simulink model "ASM_Traffic_A11"  (R2026a)
settings: Solver=ode1  StartTime=SIM.tstart.v  StopTime=SIM.tend.v  FixedStep=SIM.StepSize.v
PostLoadFcn:
  | if any(exist('dsrtsu_mdlpostloadfcn', 'file') ~= 0), dsrtsu_mdlpostloadfcn('Execute', bdroot); end
  | try, asm_mdl_postloadfcn(bdroot, 'UpdateModel', 3600); catch, disp(lasterr); end,
InitFcn:
  | , if any(exist('rtifpga_mdlclblib', 'file') ~= 0), rtifpga_mdlclblib('Init', bdroot); end,
  | , if any(exist('dsmpb_private', 'file') ~= 0), dsmpb_private('dsmpb_mdlclblib', 'Init', bdroot); end,
undefined symbols (not defined in the file): _to_, a0b2, ASM_BrakeHydraulics_DemoSystems, ASM_VehicleDynamics_DemoSystems, b98103fe8ad365046cd0, BrakeCircuit, controllerConfig, CPT, Crankshaft, DiscIntNeverNeededParam, dsmsi, FinalDriveAssembly, instance, MDL, ModeSignals, mu, Pos_BrakePedal_Maneuver, rad, RefSignals, s_to_rpm, SIM, SoftECU, Suspension, Tire, Transmission
libraries: ASM_Traffic_lib x135, simulink x98, ASM_Utils_lib x77, ASM_VehicleDynamics_lib x70, ASM_Environment_lib x22, dsmpblib x20, dsmsilib x15, MDLD_Utils_lib x10, ASM_BrakeHydraulics_lib x3, sl_discontinuities x2
(part 11 of 63)

== system ASM_Traffic_A11/Drivetrain/Control/SoftECU_Drivetrain ==
  note: -------------
  note: Plant
  note: -------------
  note: User Interface
  note: Control
  note: -------------
  note: Inport colors:
  note: External Signals
  note: -------------
  UserInterface : Inport
  Interface_In : Inport  Port=2
  Plant : Inport  Port=3
  Bus Creator : BusCreator  Inputs=8
  Bus Selector1 : BusSelector  OutputSignals=ExternalModel.Pos_AccPedal[%],ExternalModel.SelectorLever[-3T|-2P|-1R|0N|1D],ExternalModel.Sw_TipShift[-1Down|0Off|1Up],ExternalModel.Gear_Max[0Off|1_n],ExternalModel.Reset_States[0|1],ExternalModel.Gear_Maneuver[],ExternalModel.Mode_GearClutch[1Stim|2Driver|3OpenClutch|4RefGear],ExternalModel.State_Engine[0|1|2|3|4],ExternalModel.State_StartStop[1Off|2NotReady|3Ready|4EngStopped],ExternalModel.Enable_v_Init[0|1]
  Bus Selector7 : BusSelector  OutputSignals=Drivetrain.Crankshaft.n_Engine[rad|s],Drivetrain.Transmission.OutputSignals.omega_In_Trm[rad|s],Drivetrain.Transmission.OutputSignals.omega_Out_Trm[rad|s],Drivetrain.Transmission.OutputSignals.Gear[]
  Constant{,1..3} (4 alike) : Constant  Value=0
  ModelDesk_MC_ID_SoftECU : ASM_Utils_lib/ModelDeskInterface/ModelDesk_MC  Tag=ASM_MAINCOMPONENT  Editable=off  MainComponent=SoftECU
  SoftECU_Transmission : Subsystem
  Terminator_1 : Terminator
  ASMSignalBus : Outport  VectorParamsAs1DForOutWhenUnconnected=off
  Out : Outport  Port=2  VectorParamsAs1DForOutWhenUnconnected=off
  wires:
  Bus Selector1/9 -> SoftECU_Transmission/13(State_StartStop[1Off|2NotReady|3Ready|4EngStopped])  "<State_StartStop[1Off|2NotReady|3Ready|4EngStopped]>"
  Bus Selector1/7 -> SoftECU_Transmission/11(GearClutch_Mode[1Stim|2SoftECU|3OpenClutch|4RefGear])  "<Mode_GearClutch[1Stim|2Driver|3OpenClutch|4RefGear]>"
  Bus Selector1/6 -> SoftECU_Transmission/10(Gear_Maneuver[])  "<Gear_Maneuver[]>"
  Bus Selector1/5 -> SoftECU_Transmission/9(Reset[0|1])  "<Reset_States[0|1]>"
  Bus Selector1/4 -> SoftECU_Transmission/8(Gear_Max_Maneuver[0Off|1_n])  "<Gear_Max[0Off|1_n]>"
  Bus Selector1/3 -> SoftECU_Transmission/7(TipShift[-1Down|0Off|1Up])  "<Sw_TipShift[-1Down|0Off|1Up]>"
  Bus Selector1/2 -> SoftECU_Transmission/6(SelectorLever[-3T|-2P|-1R|0N|1D])  "<SelectorLever[-3T|-2P|-1R|0N|1D]>"
  Bus Selector1/1 -> SoftECU_Transmission/5(Pos_AccPedal_Driver[%])  "<Pos_AccPedal[%]>"
  Bus Selector1/8 -> SoftECU_Transmission/12(State_Engine[0|1|2|3|4])  "<State_Engine[0|1|2|3|4]>"
  Interface_In/1 -> Bus Selector1/1
  Constant3/1 -> Bus Creator/8  "Ctrl_Clutch_4WD[0_1]"
  Constant2/1 -> Bus Creator/7  "Ctrl_RearDiff[0_1]"
  Constant1/1 -> Bus Creator/6  "Ctrl_FrontDiff[0_1]"
  Constant/1 -> Bus Creator/5  "Ctrl_CentralDiff[0_1]"
  UserInterface/1 -> Terminator_1/1
  Bus Creator/1 -> Out/1  "Drivetrain"
  SoftECU_Transmission/5(Gear[]) -> Bus Creator/4  "Gear[]"
  SoftECU_Transmission/4(Ctrl_Lockup_Clutch[0_1]) -> Bus Creator/3  "Ctrl_Lockup_Clutch[0_1]"
  SoftECU_Transmission/3(Ctrl_Parking_Pawl[0|1]) -> Bus Creator/2  "Ctrl_Parking_Pawl[0|1]"
  SoftECU_Transmission/2(Factor_Trq_Engine_Red[%]) -> Bus Creator/1  "Factor_Trq_Engine_Red[%]"
  Bus Selector7/4 -> SoftECU_Transmission/4(Gear_Current[])  "<Gear[]>"
  Bus Selector7/3 -> SoftECU_Transmission/3(omega_Out_Trm[rad|s])  "<omega_Out_Trm[rad|s]>"
  Bus Selector7/2 -> SoftECU_Transmission/2(omega_In_Trm[rad|s])  "<omega_In_Trm[rad|s]>"
  Bus Selector7/1 -> SoftECU_Transmission/1(n_Engine[rad|s])  "<n_Engine[rad|s]>"
  Plant/1 -> Bus Selector7/1
  SoftECU_Transmission/1(ASMSignalBus) -> ASMSignalBus/1
  Bus Selector1/10 -> SoftECU_Transmission/14(Enable_v_Init[0|1])  "<Enable_v_Init[0|1]>"

== system ASM_Traffic_A11/Drivetrain/Control/Sw_ECU_Signals ==
  SoftECU : Inport
  ExternalECU : Inport  Port=2
  Bus Creator4 : BusCreator  Inputs=8
  Bus Selector1 : BusSelector  OutputSignals=ExternalECU.Factor_Trq_Engine_Red[%],ExternalECU.Ctrl_Parking_Pawl[0|1],ExternalECU.Ctrl_Lockup_Clutch[0_1],ExternalECU.Gear[],ExternalECU.Ctrl_CentralDiff[0_1],ExternalECU.Ctrl_FrontDiff[0_1],ExternalECU.Ctrl_RearDiff[0_1],ExternalECU.Ctrl_Clutch_4WD[0_1]
  Bus Selector2 : BusSelector  OutputSignals=Factor_Trq_Engine_Red[%],Ctrl_Parking_Pawl[0|1],Ctrl_Lockup_Clutch[0_1],Gear[],Ctrl_CentralDiff[0_1],Ctrl_FrontDiff[0_1],Ctrl_RearDiff[0_1],Ctrl_Clutch_4WD[0_1]
  Ctrl_CentralDiff[0_1] : Subsystem
  Ctrl_Clutch_4WD[0_1] : Subsystem
  Ctrl_FrontDiff[0_1] : Subsystem
  Ctrl_Lockup_Clutch[0_1] : Subsystem
  Ctrl_Parking_Pawl[0|1] : Subsystem
  Ctrl_RearDiff[0_1] : Subsystem
  Factor_Trq_Engine_Red[%] : Subsystem
  Gear[] : Subsystem
  ECU_Signals : Outport  VectorParamsAs1DForOutWhenUnconnected=off
  wires:
  Ctrl_Clutch_4WD[0_1]/1(Ctrl_Clutch_4WD[0_1]) -> Bus Creator4/8  "Ctrl_Clutch_4WD[0_1]"
  Ctrl_RearDiff[0_1]/1(Ctrl_RearDiff[0_1]) -> Bus Creator4/7  "Ctrl_RearDiff[0_1]"
  Ctrl_FrontDiff[0_1]/1(Ctrl_FrontDiff[0_1]) -> Bus Creator4/6  "Ctrl_FrontDiff[0_1]"
  Ctrl_CentralDiff[0_1]/1(Ctrl_CentralDiff[0_1]) -> Bus Creator4/5  "Ctrl_CentralDiff[0_1]"
  Gear[]/1(Gear[]) -> Bus Creator4/4  "Gear[]"
  Ctrl_Lockup_Clutch[0_1]/1(Ctrl_Lockup_Clutch[0_1]) -> Bus Creator4/3  "Ctrl_Lockup_Clutch[0_1]"
  Ctrl_Parking_Pawl[0|1]/1(Ctrl_Parking_Pawl[0|1]) -> Bus Creator4/2  "Ctrl_Parking_Pawl[0|1]"
  Factor_Trq_Engine_Red[%]/1(Factor_Trq_Engine_Red[%]) -> Bus Creator4/1  "Factor_Trq_Engine_Red[%]"
  Bus Selector1/4 -> Gear[]/2(RealECU)  "<Gear[]>"
  Bus Selector1/5 -> Ctrl_CentralDiff[0_1]/2(RealECU)  "<Ctrl_CentralDiff[0_1]>"
  Bus Selector1/6 -> Ctrl_FrontDiff[0_1]/2(RealECU)  "<Ctrl_FrontDiff[0_1]>"
  Bus Selector1/7 -> Ctrl_RearDiff[0_1]/2(RealECU)  "<Ctrl_RearDiff[0_1]>"
  Bus Selector1/8 -> Ctrl_Clutch_4WD[0_1]/2(RealECU)  "<Ctrl_Clutch_4WD[0_1]>"
  Bus Selector1/3 -> Ctrl_Lockup_Clutch[0_1]/2(RealECU)  "<Ctrl_Lockup_Clutch[0_1]>"
  Bus Selector1/2 -> Ctrl_Parking_Pawl[0|1]/2(RealECU)  "<Ctrl_Parking_Pawl[0|1]>"
  Bus Selector1/1 -> Factor_Trq_Engine_Red[%]/2(RealECU)  "<Factor_Trq_Engine_Red[%]>"
  Bus Selector2/8 -> Ctrl_Clutch_4WD[0_1]/1(SoftECU)  "<Ctrl_Clutch_4WD[0_1]>"
  Bus Selector2/7 -> Ctrl_RearDiff[0_1]/1(SoftECU)  "<Ctrl_RearDiff[0_1]>"
  Bus Selector2/6 -> Ctrl_FrontDiff[0_1]/1(SoftECU)  "<Ctrl_FrontDiff[0_1]>"
  Bus Selector2/5 -> Ctrl_CentralDiff[0_1]/1(SoftECU)  "<Ctrl_CentralDiff[0_1]>"
  Bus Selector2/4 -> Gear[]/1(SoftECU)  "<Gear[]>"
  Bus Selector2/3 -> Ctrl_Lockup_Clutch[0_1]/1(SoftECU)  "<Ctrl_Lockup_Clutch[0_1]>"
  Bus Selector2/2 -> Ctrl_Parking_Pawl[0|1]/1(SoftECU)  "<Ctrl_Parking_Pawl[0|1]>"
  Bus Selector2/1 -> Factor_Trq_Engine_Red[%]/1(SoftECU)  "<Factor_Trq_Engine_Red[%]>"
  Bus Creator4/1 -> ECU_Signals/1  "Control"
  SoftECU/1 -> Bus Selector2/1
  ExternalECU/1 -> Bus Selector1/1

== system ASM_Traffic_A11/Drivetrain/Control/UserInterface ==
  note: Drivetrain Control
  In : Inport
  ASMSignalBus_Control : Subsystem
  DISP_Control : Subsystem
  PAR_Control : Subsystem
  Out : Outport  VectorParamsAs1DForOutWhenUnconnected=off
  wires:
  PAR_Control/1(Out) -> Out/1
  In/1 -> DISP_Control/1(In), ASMSignalBus_Control/1(In)

== system ASM_Traffic_A11/Drivetrain/Interface_In/ExternalSignals ==
  Enable : EnablePort
  ExternalECU_Transmission : Subsystem
  ExternalECU_Transmission_In : dsmpblib/Data Inport  Tag=ASM_MPB  Priority=10000
      settings: SourceProductName=dSPACE Model Interface Package for Simulink (MIPS)
  ExternalECU_Transmission_Out : Outport
  wires:
  ExternalECU_Transmission/1(Out) -> ExternalECU_Transmission_Out/1
  ExternalECU_Transmission_In/8 -> ExternalECU_Transmission/8(Ctrl_Clutch_4WD[0_1])
  ExternalECU_Transmission_In/7 -> ExternalECU_Transmission/7(Ctrl_RearDiff[0_1])
  ExternalECU_Transmission_In/6 -> ExternalECU_Transmission/6(Ctrl_FrontDiff[0_1])
  ExternalECU_Transmission_In/5 -> ExternalECU_Transmission/5(Ctrl_CentralDiff[0_1])
  ExternalECU_Transmission_In/4 -> ExternalECU_Transmission/4(Gear[])
  ExternalECU_Transmission_In/3 -> ExternalECU_Transmission/3(Ctrl_Lockup_Clutch[0_1])
  ExternalECU_Transmission_In/2 -> ExternalECU_Transmission/2(Ctrl_Parking_Pawl[0|1])
  ExternalECU_Transmission_In/1 -> ExternalECU_Transmission/1(Factor_Trq_Engine_Red[%])

== system ASM_Traffic_A11/Drivetrain/Interface_In/ModelSignals ==
  Sw_ModelPortBlocks[0Disabled|1Enabled] : Inport
  Sw_ModelDeskPlottingInterface[0Disabled|1Enabled] : Inport  Port=2
  n_Engine_Set[rpm] : Inport  Port=3
  Sw_Testbench[0Off|1On] : Inport  Port=4
  Pos_ClutchPedal[%] : Inport  Port=5
  Gear[] : Inport  Port=6
  Reset_States[0|1] : Inport  Port=7
  Trq_MeanEff_Engine[Nm] : Inport  Port=8
  omega_Wheel[FL;FR;RL;RR][rad|s] : Inport  Port=9
  Enable_v_Init[0|1] : Inport  Port=10
  Pos_AccPedal[%] : Inport  Port=11
  SelectorLever[-3T|-2P|-1R|0N|1D] : Inport  Port=12  PortDimensions=1
  Sw_TipShift[-1Down|0Off|1Up] : Inport  Port=13
  Gear_Maneuver[] : Inport  Port=14
  Mode_GearClutch[1Stim|2Driver|3OpenClutch|4RefGear] : Inport  Port=15
  Gear_Max[0Off|1_n] : Inport  Port=16
  State_Engine[0|1|2|3|4] : Inport  Port=17
  State_StartStop[1Off|2NotReady|3Ready|4EngStopped] : Inport  Port=18
  Sw_Starter[0|1] : Inport  Port=19
  CrankAngle_Cyl[aTDC] : Inport  Port=20
  Type_Engine_1[0Unkown|1Other|2Otto|3Diesel|4Electric] : Inport  Port=21
  Bus Creator : BusCreator  Inputs=21
  CrankAngle_Cyl[aTDC]_ : Subsystem
      mask Display: disp('')
  Enable_v_Init[0|1]_ : Subsystem
      mask Display: disp('')
  Gear[]_ : Subsystem
      mask Display: disp('')
  Gear_Maneuver[]_ : Subsystem
      mask Display: disp('')
  Gear_Max[0Off|1_n]_ : Subsystem
      mask Display: disp('')
  Mode_GearClutch[1Stim|2Driver|3OpenClutch|4RefGear]_ : Subsystem
      mask Display: disp('')
  Pos_AccPedal[%]_ : Subsystem
      mask Display: disp('')
  Pos_ClutchPedal[%]_ : Subsystem
      mask Display: disp('')
  Reset_States[0|1]_ : Subsystem
      mask Display: disp('')
  SelectorLever[-3T|-2P|-1R|0N|1D]_ : Subsystem
      mask Display: disp('')
  State_Engine[0|1|2|3|4]_ : Subsystem
      mask Display: disp('')
  State_StartStop[1Off|2NotReady|3Ready|4EngStopped]_ : Subsystem
      mask Display: disp('')
  Sw_ModelDeskPlottingInterface[0Disabled|1Enabled]_ : Subsystem
  Sw_ModelPortBlocks[0Disabled|1Enabled]_ : Subsystem
  Sw_Starter[0|1]_ : Subsystem
      mask Display: disp('')
  Sw_Testbench[0Off|1On]_ : Subsystem
      mask Display: disp('')
  Sw_TipShift[-1Down|0Off|1Up]_ : Subsystem
      mask Display: disp('')
  Trq_MeanEff_Engine[Nm]_ : Subsystem
      mask Display: disp('')
  Type_Engine_1[0Unkown|1Other|2Otto|3Diesel|4Electric]_ : Subsystem
      mask Display: disp('')
  n_Engine_Set[rpm]_ : Subsystem
      mask Display: disp('')
  omega_Wheel[FL;FR;RL;RR][rad|s]_ : Subsystem
      mask Display: disp('')
  Out : Outport  VectorParamsAs1DForOutWhenUnconnected=off
  wires:
  Sw_ModelDeskPlottingInterface[0Disabled|1Enabled]_/1(Out1) -> Bus Creator/2  "Sw_ModelDeskPlottingInterface[0Disabled|1Enabled]"
  Sw_ModelPortBlocks[0Disabled|1Enabled]_/1(Out1) -> Bus Creator/1  "Sw_ModelPortBlocks[0Disabled|1Enabled]"
  Sw_ModelDeskPlottingInterface[0Disabled|1Enabled]/1 -> Sw_ModelDeskPlottingInterface[0Disabled|1Enabled]_/1(In1)
  Sw_ModelPortBlocks[0Disabled|1Enabled]/1 -> Sw_ModelPortBlocks[0Disabled|1Enabled]_/1(In1)
  Bus Creator/1 -> Out/1  "ExternalModel"
  Pos_ClutchPedal[%]_/1(Out1) -> Bus Creator/5  "Pos_ClutchPedal[%]"
  Gear[]_/1(Out1) -> Bus Creator/6  "Gear[]"
  Gear[]/1 -> Gear[]_/1(In1)
  Pos_ClutchPedal[%]/1 -> Pos_ClutchPedal[%]_/1(In1)
  Sw_Testbench[0Off|1On]_/1(Out1) -> Bus Creator/4  "Sw_Testbench[0Off|1On]"
  Sw_Testbench[0Off|1On]/1 -> Sw_Testbench[0Off|1On]_/1(In1)
  n_Engine_Set[rpm]_/1(Out1) -> Bus Creator/3  "n_Engine_Set[rpm]"
  n_Engine_Set[rpm]/1 -> n_Engine_Set[rpm]_/1(In1)
  Reset_States[0|1]_/1(Out1) -> Bus Creator/7  "Reset_States[0|1]"
  Reset_States[0|1]/1 -> Reset_States[0|1]_/1(In1)
  Trq_MeanEff_Engine[Nm]_/1(Out1) -> Bus Creator/8  "Trq_MeanEff_Engine[Nm]"
  Trq_MeanEff_Engine[Nm]/1 -> Trq_MeanEff_Engine[Nm]_/1(In1)
  omega_Wheel[FL;FR;RL;RR][rad|s]_/1(Out1) -> Bus Creator/9  "omega_Wheel[FL;FR;RL;RR][rad|s]"
  omega_Wheel[FL;FR;RL;RR][rad|s]/1 -> omega_Wheel[FL;FR;RL;RR][rad|s]_/1(In1)
  Enable_v_Init[0|1]/1 -> Enable_v_Init[0|1]_/1(In1)
  Enable_v_Init[0|1]_/1(Out1) -> Bus Creator/10  "Enable_v_Init[0|1]"
  Sw_TipShift[-1Down|0Off|1Up]_/1(Out1) -> Bus Creator/13  "Sw_TipShift[-1Down|0Off|1Up]"
  Gear_Maneuver[]_/1(Out1) -> Bus Creator/14  "Gear_Maneuver[]"
  Pos_AccPedal[%]/1 -> Pos_AccPedal[%]_/1(In1)
  SelectorLever[-3T|-2P|-1R|0N|1D]/1 -> SelectorLever[-3T|-2P|-1R|0N|1D]_/1(In1)
  Mode_GearClutch[1Stim|2Driver|3OpenClutch|4RefGear]_/1(Out1) -> Bus Creator/15  "Mode_GearClutch[1Stim|2Driver|3OpenClutch|4RefGear]"
  Mode_GearClutch[1Stim|2Driver|3OpenClutch|4RefGear]/1 -> Mode_GearClutch[1Stim|2Driver|3OpenClutch|4RefGear]_/1(In1)
  Gear_Max[0Off|1_n]/1 -> Gear_Max[0Off|1_n]_/1(In1)
  Gear_Maneuver[]/1 -> Gear_Maneuver[]_/1(In1)
  Gear_Max[0Off|1_n]_/1(Out1) -> Bus Creator/16  "Gear_Max[0Off|1_n]"
  State_Engine[0|1|2|3|4]_/1(Out1) -> Bus Creator/17  "State_Engine[0|1|2|3|4]"
  Sw_TipShift[-1Down|0Off|1Up]/1 -> Sw_TipShift[-1Down|0Off|1Up]_/1(In1)
  State_StartStop[1Off|2NotReady|3Ready|4EngStopped]_/1(Out1) -> Bus Creator/18  "State_StartStop[1Off|2NotReady|3Ready|4EngStopped]"
  SelectorLever[-3T|-2P|-1R|0N|1D]_/1(Out1) -> Bus Creator/12  "SelectorLever[-3T|-2P|-1R|0N|1D]"
  Pos_AccPedal[%]_/1(Out1) -> Bus Creator/11  "Pos_AccPedal[%]"
  State_StartStop[1Off|2NotReady|3Ready|4EngStopped]/1 -> State_StartStop[1Off|2NotReady|3Ready|4EngStopped]_/1(In1)
  State_Engine[0|1|2|3|4]/1 -> State_Engine[0|1|2|3|4]_/1(In1)
  Sw_Starter[0|1]/1 -> Sw_Starter[0|1]_/1(In1)
  CrankAngle_Cyl[aTDC]/1 -> CrankAngle_Cyl[aTDC]_/1(In1)
  CrankAngle_Cyl[aTDC]_/1(Out1) -> Bus Creator/20  "CrankAngle_Cyl[aTDC]"
  Sw_Starter[0|1]_/1(Out1) -> Bus Creator/19  "Sw_Starter[0|1]"
  Type_Engine_1[0Unkown|1Other|2Otto|3Diesel|4Electric]_/1(Out1) -> Bus Creator/21  "Type_Engine_1[0Unkown|1Other|2Otto|3Diesel|4Electric]"
  Type_Engine_1[0Unkown|1Other|2Otto|3Diesel|4Electric]/1 -> Type_Engine_1[0Unkown|1Other|2Otto|3Diesel|4Electric]_/1(In1)

== system ASM_Traffic_A11/Drivetrain/Interface_Out/Animation ==
  n_Engine[rpm] : Inport
  Gear[] : Inport  Port=2
  BusCreator : BusCreator  Inputs=2
  Gear[]_ : Subsystem
      mask Display: disp('')
  n_Engine[rpm]_ : Subsystem
      mask Display: disp('')
  Out : Outport  VectorParamsAs1DForOutWhenUnconnected=off
  wires:
  BusCreator/1 -> Out/1  "Animation"
  n_Engine[rpm]_/1(Out1) -> BusCreator/1  "n_Engine[rpm]"
  Gear[]_/1(Out1) -> BusCreator/2  "Gear[]"
  n_Engine[rpm]/1 -> n_Engine[rpm]_/1(In1)
  Gear[]/1 -> Gear[]_/1(In1)

== system ASM_Traffic_A11/Drivetrain/Interface_Out/Control_ModelSignals ==
  Factor_Trq_Engine_Red[%] : Inport
  Ctrl_Parking_Pawl[0|1] : Inport  Port=2
  Bus Creator : BusCreator  Inputs=2
  Ctrl_Parking_Pawl[0|1]_ : Subsystem
      mask Display: disp('')
  Factor_Trq_Engine_Red[%]_ : Subsystem
      mask Display: disp('')
  Out : Outport  VectorParamsAs1DForOutWhenUnconnected=off
  wires:
  Factor_Trq_Engine_Red[%]/1 -> Factor_Trq_Engine_Red[%]_/1(In1)
  Bus Creator/1 -> Out/1  "Control"
  Factor_Trq_Engine_Red[%]_/1(Out1) -> Bus Creator/1  "Factor_Trq_Engine_Red[%]"
  Ctrl_Parking_Pawl[0|1]_/1(Out1) -> Bus Creator/2  "Ctrl_Parking_Pawl[0|1]"
  Ctrl_Parking_Pawl[0|1]/1 -> Ctrl_Parking_Pawl[0|1]_/1(In1)

== system ASM_Traffic_A11/Drivetrain/Interface_Out/Plant_ModelSignals ==
  n_Engine[rpm] : Inport
  omega_Out_Trm[rad|s] : Inport  Port=2
  Gear[] : Inport  Port=3
  i_FinalDrive[] : Inport  Port=4
  i_FrontDrive[] : Inport  Port=5
  i_RearDrive[] : Inport  Port=6
  TrqDistri_Front_Rear[0_1] : Inport  Port=7
  Trq_Out_Front_Diff[Nm] : Inport  Port=8
  Trq_Shaft[FL;FR;RL;RR][Nm] : Inport  Port=9
  i_unsync_Trm[] : Inport  Port=10
  Sw_CrankShaft_Reset[0Disabled|1Enabled] : Inport  Port=11
  Mode_Transmission[1Manual|2Automatic] : Inport  Port=12
  Mode_Drivetrain[1|2|3|4|5] : Inport  Port=13
  Type_Engine_1[0Unkown|1Other|2Otto|3Diesel|4Electric] : Inport  Port=14
  Trq_Engine_1[Nm] : Inport  Port=15
  n_Engine_1[rpm] : Inport  Port=16
  Type_Engine_2[0Unkown|1Other|2Otto|3Diesel|4Electric] : Inport  Port=17
  Trq_Engine_2[Nm] : Inport  Port=18
  n_Engine_2[rpm] : Inport  Port=19
  Trq_BSG[Nm] : Inport  Port=20
  Bus Creator : BusCreator  Inputs=20
  Gear[]_ : Subsystem
      mask Display: disp('')
  Mode_Drivetrain[1|2|3|4|5]_ : Subsystem
      mask Display: disp('')
  Mode_Transmission[1Manual|2Automatic]_ : Subsystem
      mask Display: disp('')
  Sw_CrankShaft_Reset[0Disabled|1Enabled]_ : Subsystem
      mask Display: disp('')
  TrqDistri_Front_Rear[0_1]_ : Subsystem
      mask Display: disp('')
  Trq_BSG[Nm]_ : Subsystem
      mask Display: disp('')
  Trq_Engine_1[Nm]_ : Subsystem
      mask Display: disp('')
  Trq_Engine_2[Nm]_ : Subsystem
      mask Display: disp('')
  Trq_Out_Front_Diff[Nm]_ : Subsystem
      mask Display: disp('')
  Trq_Shaft[FL;FR;RL;RR][Nm]_ : Subsystem
      mask Display: disp('')
  Type_Engine_1[0Unkown|1Other|2Otto|3Diesel|4Electric]_ : Subsystem
      mask Display: disp('')
  Type_Engine_2[0Unkown|1Other|2Otto|3Diesel|4Electric]_ : Subsystem
      mask Display: disp('')
  i_FinalDrive[]_ : Subsystem
      mask Display: disp('')
  i_FrontDrive[]_ : Subsystem
      mask Display: disp('')
  i_RearDrive[]_ : Subsystem
      mask Display: disp('')
  i_unsync_Trm[]_ : Subsystem
      mask Display: disp('')
  n_Engine[rpm]_ : Subsystem
      mask Display: disp('')
  n_Engine_1[rpm]_ : Subsystem
      mask Display: disp('')
  n_Engine_2[rpm]_ : Subsystem
      mask Display: disp('')
  omega_Out_Trm[rad|s]_ : Subsystem
      mask Display: disp('')
  Out : Outport  VectorParamsAs1DForOutWhenUnconnected=off
  wires:
  n_Engine_2[rpm]_/1(Out1) -> Bus Creator/19  "n_Engine_2[rpm]"
  n_Engine_2[rpm]/1 -> n_Engine_2[rpm]_/1(In1)
  n_Engine_1[rpm]_/1(Out1) -> Bus Creator/16  "n_Engine_1[rpm]"
  n_Engine_1[rpm]/1 -> n_Engine_1[rpm]_/1(In1)
  Bus Creator/1 -> Out/1  "Plant"
  i_RearDrive[]_/1(Out1) -> Bus Creator/6  "i_RearDrive[]"
  i_RearDrive[]/1 -> i_RearDrive[]_/1(In1)
  i_FrontDrive[]_/1(Out1) -> Bus Creator/5  "i_FrontDrive[]"
  i_FrontDrive[]/1 -> i_FrontDrive[]_/1(In1)
  TrqDistri_Front_Rear[0_1]/1 -> TrqDistri_Front_Rear[0_1]_/1(In1)
  TrqDistri_Front_Rear[0_1]_/1(Out1) -> Bus Creator/7  "TrqDistri_Front_Rear[0_1]"
  i_unsync_Trm[]/1 -> i_unsync_Trm[]_/1(In1)
  i_unsync_Trm[]_/1(Out1) -> Bus Creator/10  "i_unsync_Trm[]"
  i_FinalDrive[]_/1(Out1) -> Bus Creator/4  "i_FinalDrive[]"
  i_FinalDrive[]/1 -> i_FinalDrive[]_/1(In1)
  omega_Out_Trm[rad|s]/1 -> omega_Out_Trm[rad|s]_/1(In1)
  n_Engine[rpm]/1 -> n_Engine[rpm]_/1(In1)
  Trq_Shaft[FL;FR;RL;RR][Nm]/1 -> Trq_Shaft[FL;FR;RL;RR][Nm]_/1(In1)
  Trq_Out_Front_Diff[Nm]/1 -> Trq_Out_Front_Diff[Nm]_/1(In1)
  n_Engine[rpm]_/1(Out1) -> Bus Creator/1  "n_Engine[rpm]"
  omega_Out_Trm[rad|s]_/1(Out1) -> Bus Creator/2  "omega_Out_Trm[rad|s]"
  Trq_Shaft[FL;FR;RL;RR][Nm]_/1(Out1) -> Bus Creator/9  "Trq_Shaft[FL;FR;RL;RR][Nm]"
  Trq_Out_Front_Diff[Nm]_/1(Out1) -> Bus Creator/8  "Trq_Out_Front_Diff[Nm]"
  Gear[]/1 -> Gear[]_/1(In1)
  Gear[]_/1(Out1) -> Bus Creator/3  "Gear[]"
  Sw_CrankShaft_Reset[0Disabled|1Enabled]_/1(Out1) -> Bus Creator/11  "Sw_CrankShaft_Reset[0Disabled|1Enabled]"
  Sw_CrankShaft_Reset[0Disabled|1Enabled]/1 -> Sw_CrankShaft_Reset[0Disabled|1Enabled]_/1(In1)
  Mode_Drivetrain[1|2|3|4|5]_/1(Out1) -> Bus Creator/13  "Mode_Drivetrain[1|2|3|4|5]"
  Mode_Transmission[1Manual|2Automatic]/1 -> Mode_Transmission[1Manual|2Automatic]_/1(In1)
  Mode_Drivetrain[1|2|3|4|5]/1 -> Mode_Drivetrain[1|2|3|4|5]_/1(In1)
  Mode_Transmission[1Manual|2Automatic]_/1(Out1) -> Bus Creator/12  "Mode_Transmission[1Manual|2Automatic]"
  Trq_BSG[Nm]/1 -> Trq_BSG[Nm]_/1(In1)
  Trq_BSG[Nm]_/1(Out1) -> Bus Creator/20  "Trq_BSG[Nm]"
  Type_Engine_1[0Unkown|1Other|2Otto|3Diesel|4Electric]/1 -> Type_Engine_1[0Unkown|1Other|2Otto|3Diesel|4Electric]_/1(In1)
  Type_Engine_1[0Unkown|1Other|2Otto|3Diesel|4Electric]_/1(Out1) -> Bus Creator/14  "Type_Engine_1[0Unkown|1Other|2Otto|3Diesel|4Electric]"
  Type_Engine_2[0Unkown|1Other|2Otto|3Diesel|4Electric]/1 -> Type_Engine_2[0Unkown|1Other|2Otto|3Diesel|4Electric]_/1(In1)
  Type_Engine_2[0Unkown|1Other|2Otto|3Diesel|4Electric]_/1(Out1) -> Bus Creator/17  "Type_Engine_2[0Unkown|1Other|2Otto|3Diesel|4Electric]"
  Trq_Engine_1[Nm]/1 -> Trq_Engine_1[Nm]_/1(In1)
  Trq_Engine_1[Nm]_/1(Out1) -> Bus Creator/15  "Trq_Engine_1[Nm]"
  Trq_Engine_2[Nm]_/1(Out1) -> Bus Creator/18  "Trq_Engine_2[Nm]"
  Trq_Engine_2[Nm]/1 -> Trq_Engine_2[Nm]_/1(In1)

== system ASM_Traffic_A11/Drivetrain/Plant/Drivetrain ==
  note: -------------
  note: Inport colors:
  note: External Signals
  note: -------------
  note: User Interface
  note: -------------
  note: -------------
  note: Control
  note: Plant
  UserInterface : Inport
  Interface_In : Inport  Port=2
  Control : Inport  Port=3
  ASMSignalCollector : Subsystem
  Bus Selector1 : BusSelector  OutputSignals=ExternalModel.n_Engine_Set[rpm],ExternalModel.Sw_Testbench[0Off|1On],ExternalModel.Reset_States[0|1],ExternalModel.Sw_Starter[0|1]
  Bus Selector2 : BusSelector  OutputSignals=Ctrl_Lockup_Clutch[0_1],Gear[]  OutputAsBus=on
  Bus Selector4 : BusSelector  OutputSignals=Mode_Drivetrain[1AWD|2FWD|3RWD|4FF-4WD|5FF]
  Bus Selector5 : BusSelector  OutputSignals=Ctrl_Parking_Pawl[0|1],Ctrl_CentralDiff[0_1],Ctrl_FrontDiff[0_1],Ctrl_RearDiff[0_1],Ctrl_Clutch_4WD[0_1]  OutputAsBus=on
  Bus Selector6 : BusSelector  OutputSignals=ExternalModel.Pos_ClutchPedal[%],ExternalModel.Gear[],ExternalModel.Enable_v_Init[0|1]
  Bus Selector7 : BusSelector  OutputSignals=Sw_CrankShaft_Reset[0Disabled|1Enabled],Mode_Transmission[1Manual|2Automatic]
  Bus Selector8 : BusSelector  OutputSignals=ExternalModel.CrankAngle_Cyl[aTDC],ExternalModel.Trq_MeanEff_Engine[Nm],ExternalModel.Reset_States[0|1]
  Bus Selector9 : BusSelector  OutputSignals=ExternalModel.omega_Wheel[FL;FR;RL;RR][rad|s],ExternalModel.Reset_States[0|1]
  Crankshaft : Subsystem  Tag=VehicleDynamics_Crankshaft
  DisableReset : Subsystem
      mask Display: disp('DisableReset')
  External_Loads : Subsystem
  Final_Drive_Assembly : Subsystem  Tag=VehicleDynamics_FinalDriveAssembly
  Goto Tag Visibility1 : GotoTagVisibility  GotoTag=ASMBUS_Drivetrain_TestBench
  Goto Tag Visibility2 : GotoTagVisibility  GotoTag=ASMBUS_Drivetrain_Starter
  Goto Tag Visibility3 : GotoTagVisibility  GotoTag=ASMBUS_Drivetrain_Crankshaft
  Goto Tag Visibility4 : GotoTagVisibility  GotoTag=ASMBUS_Drivetrain_FinalDriveAssembly
  Goto Tag Visibility5 : GotoTagVisibility  GotoTag=ASMBUS_Drivetrain_Transmission
  ModelDesk_MC_ID_Drivetrain : ASM_Utils_lib/ModelDeskInterface/ModelDesk_MC  Tag=ASM_MAINCOMPONENT  Editable=off  MainComponent=Drivetrain
  OpenCrankshaft : ASM_Utils_lib/Miscellaneous/OpenSystem  popupLibBlk=<select here>  popupTargetDemo=<select here>  Demosystem=VehicleDynamics_Crankshaft  variantLib=ASM_VehicleDynamics_DemoSystems/Crankshaft
  OpenFinalDriveAssembly : ASM_Utils_lib/Miscellaneous/OpenSystem  popupLibBlk=<select here>  popupTargetDemo=<select here>  Demosystem=VehicleDynamics_FinalDriveAssembly  variantLib=ASM_VehicleDynamics_DemoSystems/FinalDriveAssembly
  OpenTransmission : ASM_Utils_lib/Miscellaneous/OpenSystem  popupLibBlk=<select here>  popupTargetDemo=<select here>  Demosystem=VehicleDynamics_Transmission  variantLib=ASM_VehicleDynamics_DemoSystems/Transmission
  STARTER : ASM_VehicleDynamics_lib/Drivetrain/Crankshaft_and_Starter/STARTER  Tag=ASM_SUBCOMPONENT  Const_Trq_n0=MDL.Drivetrain.Starter.Const_Trq_n0  Const_n_Trq0=MDL.Drivetrain.Starter.Const_n_Trq0  Const_Inertia_Starter=MDL.Drivetrain.Starter.Const_Inertia_Starter  ASMProperties=struct('Name','STARTER','Version','4.0','Library','ASM_VehicleDynamics_lib')  ASMInstanceName=starter  ASMInstanceID=1
  TEST_BENCH : ASM_VehicleDynamics_lib/Drivetrain/Crankshaft_and_Starter/TEST_BENCH  Tag=ASM_SUBCOMPONENT  Const_P_Gain=MDL.Drivetrain.TestBench.Const_P_Gain  Const_I_Gain=MDL.Drivetrain.TestBench.Const_I_Gain  Const_Trq_Max_TestBench=MDL.Drivetrain.TestBench.Const_Trq_Max_TestBench  Const_Inertia_TestBench=MDL.Drivetrain.TestBench.Const_Inertia_TestBench  StepSize=SIM.StepSize  ASMProperties=struct('Name','TEST_BENCH','Version','2.0','Library','ASM_VehicleDynamics_lib')  ASMInstanceName=test_bench  ASMInstanceID=1
  Terminator : Terminator
  Transmission : Subsystem  Tag=VehicleDynamics_Transmission
  ASMSignalBus : Outport  VectorParamsAs1DForOutWhenUnconnected=off
  tag scope: ASMBUS_Drivetrain_Starter=scoped, ASMBUS_Drivetrain_TestBench=scoped
  wires:
  External_Loads/2(Trq_External[Nm]) -> Crankshaft/3(Trq_External[Nm])
  External_Loads/1(Inertia_External[kgm2]) -> Crankshaft/2(Inertia_External[kgm2])
  Bus Selector2/1 -> Transmission/8(ECU_Signals)
  Bus Selector7/2 -> Transmission/4(Mode_Transmission[1|2])  "<Mode_Transmission[1Manual|2Automatic]>"
  Bus Selector9/2 -> Final_Drive_Assembly/5(Reset[0|1])  "<Reset_States[0|1]>"
  Bus Selector9/1 -> Final_Drive_Assembly/4(omega_Wheel[FL,FR,RL,RR][rad|s])  "<omega_Wheel[FL;FR;RL;RR][rad|s]>"
  Bus Selector6/2 -> Transmission/6(Gear_MT[])  "<Gear[]>"
  Bus Selector6/1 -> Transmission/5(Pos_ClutchPedal_MT[%])  "<Pos_ClutchPedal[%]>"
  Bus Selector7/1 -> DisableReset/2(Sw_CrankShaft_Reset[0Disabled|1Enabled])  "<Sw_CrankShaft_Reset[0Disabled|1Enabled]>"
  Bus Selector8/1 -> Crankshaft/4(CrankAngle_Cyl[deg])  "<CrankAngle_Cyl[aTDC]>"
  Bus Selector1/4 -> STARTER/1  "<Sw_Starter[0|1]>"
  Bus Selector1/3 -> TEST_BENCH/4  "<Reset_States[0|1]>"
  Bus Selector1/2 -> TEST_BENCH/3  "<Sw_Testbench[0Off|1On]>"
  Bus Selector1/1 -> TEST_BENCH/2  "<n_Engine_Set[rpm]>"
  Bus Selector4/1 -> Final_Drive_Assembly/6(Mode_Drivetrain[1|2|3|4|5])  "<Mode_Drivetrain[1AWD|2FWD|3RWD|4FF-4WD|5FF]>"
  Bus Selector5/1 -> Final_Drive_Assembly/3(ECU_Signals)
  ASMSignalCollector/1(ASMSignalBus) -> ASMSignalBus/1
  Control/1 -> Bus Selector5/1, Bus Selector2/1
  Bus Selector8/3 -> DisableReset/1(Reset_States[0|1])  "<Reset_States[0|1]>"
  Bus Selector8/2 -> Crankshaft/5(Trq_Engine[Nm]), Transmission/3(Trq_Engine[Nm])  "<Trq_MeanEff_Engine[Nm]>"
  Interface_In/1 -> Bus Selector6/1, Bus Selector9/1, Bus Selector8/1, ASMSignalCollector/1(Interface_In), Bus Selector1/1
  UserInterface/1 -> External_Loads/4(UserInterface), Bus Selector4/1, Bus Selector7/1
  TEST_BENCH/2 -> Crankshaft/1(Trq_TestBench[Nm])
  Crankshaft/1(n_Engine[rpm]) -> STARTER/2, TEST_BENCH/1
  Final_Drive_Assembly/2(Trq_Shaft[FL,FR,RL,RR][Nm]) -> Terminator/1
  TEST_BENCH/3 -> External_Loads/1(Inertia_TestBench[kgm2])
  Crankshaft/2(n_Engine[rad|s]) -> Transmission/1(n_Engine[rad|s])
  DisableReset/1(Reset[0|1]) -> Crankshaft/6(Reset[0|1]), Transmission/2(Reset[0|1])
  STARTER/1 -> [ASMBUS_Drivetrain_Starter]
  Transmission/1(Trq_Fric[Nm]) -> Crankshaft/7(Trq_Fric_Clutch[Nm])
  Transmission/3(Inertia_Out_Trm[kgm2]) -> Final_Drive_Assembly/1(Inertia_Trm[kgm2])
  STARTER/2 -> External_Loads/2(Trq_Starter[Nm])
  Transmission/4(Trq_Out_Trm[Nm]) -> Final_Drive_Assembly/2(Trq_Out_Trm[Nm])
  TEST_BENCH/1 -> [ASMBUS_Drivetrain_TestBench]
  Final_Drive_Assembly/1(omega_In_Diff[rad|s]) -> Transmission/9(omega_In_Diff[rad|s])
  STARTER/3 -> External_Loads/3(Inertia_Starter[kgm2])
  Bus Selector6/3 -> Transmission/7(Enable_v_Init[0|1])  "<Enable_v_Init[0|1]>"
  Transmission/2(omega_In_Trm[rad|s]) -> Crankshaft/8(omega_In_Trm[rad|s])

== system ASM_Traffic_A11/Drivetrain/Plant/UserInterface ==
  note: Drivetrain
  In : Inport
  ASMSignalBus_Plant : Subsystem
  DISP_Plant : Subsystem
  PAR_Plant : Subsystem
  Out : Outport  VectorParamsAs1DForOutWhenUnconnected=off
  wires:
  PAR_Plant/1(Out) -> Out/1
  In/1 -> ASMSignalBus_Plant/1(In), DISP_Plant/1(In)

== system ASM_Traffic_A11/Drivetrain/SignalInterface/ASMSignalInterface ==
  ASMSignalBus : Inport
  Enable : EnablePort
  signal_structure : Subsystem
  wires:
  ASMSignalBus/1 -> signal_structure/1(ASMSignalBus)

== system ASM_Traffic_A11/Drivetrain/SignalInterface/ExternalOutports ==
  In1 : Inport
  Enable : EnablePort
  Drivetrain : dsmpblib/Data Outport  Tag=ASM_MPB  Priority=-10000
      settings: SourceProductName=dSPACE Model Interface Package for Simulink (MIPS)
  Select_Outport_Signals : Subsystem
  wires:
  In1/1 -> Select_Outport_Signals/1(ASMSignalBus)
  Select_Outport_Signals/5(FinalDriveAssembly) -> Drivetrain/5
  Select_Outport_Signals/4(Transmission) -> Drivetrain/4
  Select_Outport_Signals/3(TestBench) -> Drivetrain/3
  Select_Outport_Signals/2(Starter) -> Drivetrain/2
  Select_Outport_Signals/1(Crankshaft) -> Drivetrain/1

== system ASM_Traffic_A11/ElectricalSystem/Control/SoftECU_ElectricalSystem ==
  UserInterface : Inport
  Interface_In : Inport  Port=2
  Plant : Inport  Port=3
  Bus Creator : BusCreator  Inputs=2
  Bus Creator1 : BusCreator  Inputs=2
  Bus Selector3 : BusSelector  OutputSignals=Battery_HV.SOC_Bat[%]
  Signal Specification : SignalSpecification
  Signal Specification1 : SignalSpecification
  Terminator : Terminator
  Terminator1 : Terminator
  ASMSignalBus : Outport  VectorParamsAs1DForOutWhenUnconnected=off
  Out : Outport  Port=2  VectorParamsAs1DForOutWhenUnconnected=off
  wires:
  UserInterface/1 -> Terminator/1
  Interface_In/1 -> Terminator1/1
  Bus Creator1/1 -> ASMSignalBus/1  "SoftECU_ElectricalSystem"
  Bus Creator/1 -> Out/1  "Control"
  Signal Specification1/1 -> Bus Creator1/2, Bus Creator/2  "SOC_Estimated_Mean[%]"
  Plant/1 -> Bus Selector3/1
  Signal Specification/1 -> Bus Creator1/1, Bus Creator/1  "SOC_Estimated_Max[%]"
  Bus Selector3/1 -> Signal Specification/1, Signal Specification1/1  "<SOC_Bat[%]>"

== system ASM_Traffic_A11/ElectricalSystem/Control/UserInterface ==
  note: Electrical System Basic Control
  In : Inport
  ASMSignalBus_Control : Subsystem
  DISP_Control : Subsystem
  PAR_Control : Subsystem
  Out : Outport  VectorParamsAs1DForOutWhenUnconnected=off
  wires:
  In/1 -> ASMSignalBus_Control/1(In), DISP_Control/1(In)
  PAR_Control/1(Out) -> Out/1

== system ASM_Traffic_A11/ElectricalSystem/Interface_In/ModelSignals ==
  Sw_ModelPortBlocks[0Disabled|1Enabled] : Inport
  Sw_ModelDeskPlottingInterface[0Disabled|1Enabled] : Inport  Port=2
  Bus Creator : BusCreator  Inputs=2
  Sw_ModelDeskPlottingInterface[0Disabled|1Enabled]_ : Subsystem
  Sw_ModelPortBlocks[0Disabled|1Enabled]_ : Subsystem
  Out : Outport
  wires:
  Bus Creator/1 -> Out/1  "ExternalModel"
  Sw_ModelDeskPlottingInterface[0Disabled|1Enabled]_/1(Out1) -> Bus Creator/2  "Sw_ModelDeskPlottingInterface[0Disabled|1Enabled]"
  Sw_ModelPortBlocks[0Disabled|1Enabled]_/1(Out1) -> Bus Creator/1  "Sw_ModelPortBlocks[0Disabled|1Enabled]"
  Sw_ModelDeskPlottingInterface[0Disabled|1Enabled]/1 -> Sw_ModelDeskPlottingInterface[0Disabled|1Enabled]_/1(In1)
  Sw_ModelPortBlocks[0Disabled|1Enabled]/1 -> Sw_ModelPortBlocks[0Disabled|1Enabled]_/1(In1)

== system ASM_Traffic_A11/ElectricalSystem/Interface_Out/Control_ModelSignals ==
  SOC_Estimated_Max[%] : Inport
  SOC_Estimated_Mean[%] : Inport  Port=2
  Bus Creator : BusCreator  Inputs=2
  SOC_Estimated_Max[%]_ : Subsystem
      mask Display: disp('')
  SOC_Estimated_Mean[%]_ : Subsystem
      mask Display: disp('')
  Out : Outport  VectorParamsAs1DForOutWhenUnconnected=off
  wires:
  SOC_Estimated_Mean[%]_/1(Out1) -> Bus Creator/2  "SOC_Estimated_Mean[%]"
  SOC_Estimated_Mean[%]/1 -> SOC_Estimated_Mean[%]_/1(In1)
  SOC_Estimated_Max[%]/1 -> SOC_Estimated_Max[%]_/1(In1)
  SOC_Estimated_Max[%]_/1(Out1) -> Bus Creator/1  "SOC_Estimated_Max[%]"
  Bus Creator/1 -> Out/1  "Control"

== system ASM_Traffic_A11/ElectricalSystem/Interface_Out/Plant_ModelSignals ==
  V_Bat_LV[V] : Inport
  SOC_Bat_LV[%] : Inport  Port=2
  T_Bat_LV[degC] : Inport  Port=3
  V_Bat_HV[V] : Inport  Port=4
  T_Bat_HV[degC] : Inport  Port=5
  V_DCLink[V] : Inport  Port=6
  I_DCLink[A] : Inport  Port=7
  I_DCDC_LS[A] : Inport  Port=8
  State_DCLink[0Off|1On] : Inport  Port=9
  Sw_DCLink_Reset[0Disabled|1Enabled] : Inport  Port=10
  Bus Creator : BusCreator  Inputs=10
  I_DCDC_LS[A]_ : Subsystem
      mask Display: disp('')
  I_DCLink[A]_ : Subsystem
      mask Display: disp('')
  SOC_Bat_LV[%]_ : Subsystem
      mask Display: disp('')
  State_DCLink[0Off|1On]_ : Subsystem
      mask Display: disp('')
  Sw_DCLink_Reset[0Disabled|1Enabled]_ : Subsystem
      mask Display: disp('')
  T_Bat_HV[degC]_ : Subsystem
      mask Display: disp('')
  T_Bat_LV[degC]_ : Subsystem
      mask Display: disp('')
  V_Bat_HV[V]_ : Subsystem
      mask Display: disp('')
  V_Bat_LV[V]_ : Subsystem
      mask Display: disp('')
  V_DCLink[V]_ : Subsystem
      mask Display: disp('')
  Out : Outport  VectorParamsAs1DForOutWhenUnconnected=off
  wires:
  I_DCDC_LS[A]/1 -> I_DCDC_LS[A]_/1(In1)
  I_DCDC_LS[A]_/1(Out1) -> Bus Creator/8  "I_DCDC_LS[A]"
  I_DCLink[A]/1 -> I_DCLink[A]_/1(In1)
  I_DCLink[A]_/1(Out1) -> Bus Creator/7  "I_DCLink[A]"
  V_DCLink[V]/1 -> V_DCLink[V]_/1(In1)
  V_Bat_HV[V]/1 -> V_Bat_HV[V]_/1(In1)
  V_Bat_LV[V]/1 -> V_Bat_LV[V]_/1(In1)
  Bus Creator/1 -> Out/1  "Plant"
  SOC_Bat_LV[%]/1 -> SOC_Bat_LV[%]_/1(In1)
  T_Bat_LV[degC]/1 -> T_Bat_LV[degC]_/1(In1)
  T_Bat_HV[degC]/1 -> T_Bat_HV[degC]_/1(In1)
  SOC_Bat_LV[%]_/1(Out1) -> Bus Creator/2  "SOC_Bat_LV[%]"
  V_Bat_LV[V]_/1(Out1) -> Bus Creator/1  "V_Bat_LV[V]"
  T_Bat_LV[degC]_/1(Out1) -> Bus Creator/3  "T_Bat_LV[degC]"
  V_Bat_HV[V]_/1(Out1) -> Bus Creator/4  "V_Bat_HV[V]"
  T_Bat_HV[degC]_/1(Out1) -> Bus Creator/5  "T_Bat_HV[degC]"
  V_DCLink[V]_/1(Out1) -> Bus Creator/6  "V_DCLink[V]"
  State_DCLink[0Off|1On]_/1(Out1) -> Bus Creator/9  "State_DCLink[0Off|1On]"
  State_DCLink[0Off|1On]/1 -> State_DCLink[0Off|1On]_/1(In1)
  Sw_DCLink_Reset[0Disabled|1Enabled]/1 -> Sw_DCLink_Reset[0Disabled|1Enabled]_/1(In1)
  Sw_DCLink_Reset[0Disabled|1Enabled]_/1(Out1) -> Bus Creator/10  "Sw_DCLink_Reset[0Disabled|1Enabled]"

== system ASM_Traffic_A11/ElectricalSystem/Plant/ElectricalSystemBasic ==
  note: -------------
  note: Plant
  note: -------------
  note: User Interface
  note: Control
  note: -------------
  note: Inport colors:
  note: External Signals
  note: -------------
  UserInterface : Inport
  Interface_In : Inport  Port=2
  Control : Inport  Port=3
  ASMSignalCollector : Subsystem
  Battery_HV : Subsystem
  Battery_LV : Subsystem
  DCLink : Subsystem
  Goto Tag Visibility1 : GotoTagVisibility  GotoTag=ASMBUS_ElectricalSystem_Battery_HV
  Goto Tag Visibility2 : GotoTagVisibility  GotoTag=ASMBUS_ElectricalSystem_DCLink
  Goto Tag Visibility5 : GotoTagVisibility  GotoTag=ASMBUS_ElectricalSystem_Battery_LV
  Terminator_{1..9} (9 alike) : Terminator
  ASMSignalBus : Outport  VectorParamsAs1DForOutWhenUnconnected=off
  tag scope: ASMBUS_ElectricalSystem_Battery_HV=scoped, ASMBUS_ElectricalSystem_Battery_LV=scoped, ASMBUS_ElectricalSystem_DCLink=scoped
  wires:
  DCLink/2(V_DCLink[V]) -> Terminator_9/1
  DCLink/1(ASMSignalBus) -> [ASMBUS_ElectricalSystem_DCLink]
  Battery_LV/4(T_Bat[degC]) -> Terminator_8/1
  Battery_LV/3(SOC_Bat[%]) -> Terminator_7/1
  Battery_HV/4(T_Bat[degC]) -> Terminator_6/1
  Battery_HV/3(SOC_Bat[%]) -> Terminator_5/1
  Battery_HV/1(ASMSignalBus) -> [ASMBUS_ElectricalSystem_Battery_HV]
  Battery_HV/2(V_Bat[V]) -> DCLink/1(V_Bat[V])
  UserInterface/1 -> Terminator_3/1
  Battery_LV/2(V_Bat[V]) -> Terminator_2/1
  Battery_LV/1(ASMSignalBus) -> [ASMBUS_ElectricalSystem_Battery_LV]
  ASMSignalCollector/1(ASMSignalBus) -> ASMSignalBus/1
  Interface_In/1 -> Terminator_1/1
  Control/1 -> Terminator_4/1

== system ASM_Traffic_A11/ElectricalSystem/Plant/UserInterface ==
  note: Electrical System Basic
  In : Inport
  ASMSignalBus_Plant : Subsystem
  DISP_Plant : Subsystem
  PAR_Plant : Subsystem
  Out : Outport  VectorParamsAs1DForOutWhenUnconnected=off
  wires:
  In/1 -> DISP_Plant/1(In), ASMSignalBus_Plant/1(In)
  PAR_Plant/1(Out) -> Out/1

== system ASM_Traffic_A11/ElectricalSystem/SignalInterface/ASMSignalInterface ==
  ASMSignalBus : Inport
  Enable : EnablePort
  signal_structure : Subsystem
  wires:
  ASMSignalBus/1 -> signal_structure/1(ASMSignalBus)

== system ASM_Traffic_A11/Engine/Control/SoftECU_Engine ==
  UserInterface : Inport
  Interface_In : Inport  Port=2
  Plant : Inport  Port=3
  Bus Creator : BusCreator  Inputs=8
  Bus Selector3 : BusSelector  OutputSignals=Engine.Trq_Driver_Des[Nm],Engine.Trq_Driver_Ind_Des[Nm],Engine.Trq_Engine_Ind_Max[Nm]
  Bus Selector6 : BusSelector  OutputSignals=ExternalModel.Enable_Trq_Decrease_Fast_ESP[0|1],ExternalModel.Trq_Decrease_Request_Fast_ESP[Nm],ExternalModel.Enable_Trq_Increase_Fast_ESP[0|1],ExternalModel.Trq_Increase_Request_Fast_ESP[Nm],ExternalModel.Enable_Trq_Request_Extern1[0|1],ExternalModel.Trq_Request_Extern1[Nm],ExternalModel.Enable_Trq_Request_Extern2[0|1],ExternalModel.Trq_Request_Extern2[Nm],ExternalModel.Enable_n_Engine_Idle_Request[0|1],ExternalModel.n_Engine_Idle_Request[rpm],ExternalModel.n_Engine[rpm],ExternalModel.Pos_AccPedal_Driver[%],ExternalModel.Sw_Ignition[0Off|1On],ExternalModel.Sw_StarterReq[0Off|1On],ExternalModel.Reset_States[0|1],ExternalModel.Sw_CrankShaft_Reset[0Disabled|1Enabled],ExternalModel.Factor_Trq_Engine_Red[%],ExternalModel.Mode_StartButtonState[1Stim|2SoftECU],ExternalModel.State_StartButton[-1|0|1|2],ExternalModel.Trq_Request_ICE[Nm],ExternalModel.Vehicle_Topology[-2|-1|0|2]
  ModelDesk_MC_ID_SoftECU : ASM_Utils_lib/ModelDeskInterface/ModelDesk_MC  Tag=ASM_MAINCOMPONENT  Editable=off  MainComponent=SoftECU
  SoftECU_Engine : Subsystem
  Terminator_1 : Terminator
  ASMSignalBus : Outport  VectorParamsAs1DForOutWhenUnconnected=off
  Out : Outport  Port=2  VectorParamsAs1DForOutWhenUnconnected=off
  wires:
  SoftECU_Engine/9(n_Engine_Idle_Set[rpm]) -> Bus Creator/8  "n_Engine_Idle_Set[rpm]"
  SoftECU_Engine/8(State_Engine[0|1|2|3|4]) -> Bus Creator/7  "State_Engine[0|1|2|3|4]"
  SoftECU_Engine/7(Sw_Starter[0Off|1On]) -> Bus Creator/6  "Sw_Starter[0Off|1On]"
  SoftECU_Engine/6(Pos_AccPedal_Driver_Des[%]) -> Bus Creator/5  "Pos_AccPedal_Driver_Des[%]"
  SoftECU_Engine/5(Pos_AccPedal_Ctrl[%]) -> Bus Creator/4  "Pos_AccPedal_Ctrl[%]"
  SoftECU_Engine/4(Trq_Shift_Request[Nm]) -> Bus Creator/3  "Trq_Shift_Request[Nm]"
  SoftECU_Engine/3(Enable_Trq_Shift_Request[0|1]) -> Bus Creator/2  "Enable_Trq_Shift_Request[0|1]"
  SoftECU_Engine/2(Sw_Engine_Dynamics_Fast[0|1]) -> Bus Creator/1  "Sw_Engine_Dynamics_Fast[0|1]"
  Bus Selector6/9 -> SoftECU_Engine/12(Enable_n_Engine_Idle_Request[0|1])  "<Enable_n_Engine_Idle_Request[0|1]>"
  Bus Selector6/8 -> SoftECU_Engine/11(Trq_Request_Extern2[Nm])  "<Trq_Request_Extern2[Nm]>"
  Bus Selector6/7 -> SoftECU_Engine/10(Enable_Trq_Request_Extern2[0|1])  "<Enable_Trq_Request_Extern2[0|1]>"
  Bus Selector6/6 -> SoftECU_Engine/9(Trq_Request_Extern1[Nm])  "<Trq_Request_Extern1[Nm]>"
  Bus Selector6/5 -> SoftECU_Engine/8(Enable_Trq_Request_Extern1[0|1])  "<Enable_Trq_Request_Extern1[0|1]>"
  Bus Selector6/4 -> SoftECU_Engine/7(Trq_Increase_Request_Fast_ESP[Nm])  "<Trq_Increase_Request_Fast_ESP[Nm]>"
  Bus Selector6/3 -> SoftECU_Engine/6(Enable_Trq_Increase_Fast_ESP[0|1])  "<Enable_Trq_Increase_Fast_ESP[0|1]>"
  Bus Selector6/2 -> SoftECU_Engine/5(Trq_Decrease_Request_Fast_ESP[Nm])  "<Trq_Decrease_Request_Fast_ESP[Nm]>"
  Bus Selector6/1 -> SoftECU_Engine/4(Enable_Trq_Decrease_Fast_ESP[0|1])  "<Enable_Trq_Decrease_Fast_ESP[0|1]>"
  Bus Selector3/1 -> SoftECU_Engine/1(Trq_Driver_Des[Nm])  "<Trq_Driver_Des[Nm]>"
  Bus Selector3/3 -> SoftECU_Engine/3(Trq_Engine_Ind_Max[Nm])  "<Trq_Engine_Ind_Max[Nm]>"
  Bus Selector3/2 -> SoftECU_Engine/2(Trq_Driver_Ind_Des[Nm])  "<Trq_Driver_Ind_Des[Nm]>"
  SoftECU_Engine/1(ASMSignalBus) -> ASMSignalBus/1
  Interface_In/1 -> Bus Selector6/1
  Bus Creator/1 -> Out/1  "Control"
  Plant/1 -> Bus Selector3/1
  UserInterface/1 -> Terminator_1/1
  Bus Selector6/10 -> SoftECU_Engine/13(n_Engine_Idle_Request[rpm])  "<n_Engine_Idle_Request[rpm]>"
  Bus Selector6/11 -> SoftECU_Engine/14(n_Engine[rpm])  "<n_Engine[rpm]>"
  Bus Selector6/12 -> SoftECU_Engine/15(Pos_AccPedal_Driver[%])  "<Pos_AccPedal_Driver[%]>"
  Bus Selector6/13 -> SoftECU_Engine/16(Sw_Ignition[0Off|1On])  "<Sw_Ignition[0Off|1On]>"
  Bus Selector6/14 -> SoftECU_Engine/17(Sw_StarterReq[0Off|1On])  "<Sw_StarterReq[0Off|1On]>"
  Bus Selector6/15 -> SoftECU_Engine/18(Reset[0|1])  "<Reset_States[0|1]>"
  Bus Selector6/16 -> SoftECU_Engine/19(Sw_CrankShaft_Reset[0Disabled|1Enabled])  "<Sw_CrankShaft_Reset[0Disabled|1Enabled]>"
  Bus Selector6/17 -> SoftECU_Engine/20(Factor_Trq_Engine_Red[%])  "<Factor_Trq_Engine_Red[%]>"
  Bus Selector6/18 -> SoftECU_Engine/21(Mode_StartButtonState[1Stim|2SoftECU])  "<Mode_StartButtonState[1Stim|2SoftECU]>"
  Bus Selector6/19 -> SoftECU_Engine/22(State_StartButton[-1|0|1|2])  "<State_StartButton[-1|0|1|2]>"
  Bus Selector6/20 -> SoftECU_Engine/23(Trq_Request_ICE[Nm])  "<Trq_Request_ICE[Nm]>"
  Bus Selector6/21 -> SoftECU_Engine/24(Vehicle_Topology[-2|-1|0|2])  "<Vehicle_Topology[-2|-1|0|2]>"

== system ASM_Traffic_A11/Engine/Control/UserInterface ==
  note: Engine Basic Control
  In : Inport
  ASMSignalBus_Control : Subsystem
  DISP_Control : Subsystem
  PAR_Control : Subsystem
  Out : Outport  VectorParamsAs1DForOutWhenUnconnected=off
  wires:
  PAR_Control/1(Out) -> Out/1
  In/1 -> ASMSignalBus_Control/1(In), DISP_Control/1(In)

== system ASM_Traffic_A11/Engine/Interface_In/ModelSignals ==
  Sw_ModelPortBlocks[0Disabled|1Enabled] : Inport
  Sw_ModelDeskPlottingInterface[0Disabled|1Enabled] : Inport  Port=2
  Sw_Ignition[0Off|1On] : Inport  Port=3
  Sw_StarterReq[0Off|1On] : Inport  Port=4
  Factor_Trq_Engine_Red[%] : Inport  Port=5
  Enable_Trq_Decrease_Fast_ESP[0|1] : Inport  Port=6
  Trq_Decrease_Request_Fast_ESP[Nm] : Inport  Port=7
  Enable_Trq_Increase_Fast_ESP[0|1] : Inport  Port=8
  Trq_Increase_Request_Fast_ESP[Nm] : Inport  Port=9
  Enable_Trq_Request_Extern1[0|1] : Inport  Port=10
  Trq_Request_Extern1[Nm] : Inport  Port=11
  Trq_Request_ICE[Nm] : Inport  Port=12
  Pos_AccPedal_Driver[%] : Inport  Port=13
  Reset_States[0|1] : Inport  Port=14
  n_Engine[rpm] : Inport  Port=15
  State_StartButton[-1|0|1|2] : Inport  Port=16
  Vehicle_Topology[-2|-1|0|2] : Inport  Port=17
  v_x_Vehicle[km|h] : Inport  Port=18
  Sw_CrankShaft_Reset[0Disabled|1Enabled] : Inport  Port=19
  Mode_StartButtonState[1Stim|2SoftECU] : Inport  Port=20
  Enable_Trq_Request_Extern2[0|1] : Inport  Port=21
  Trq_Request_Extern2[Nm] : Inport  Port=22
  Enable_n_Engine_Idle_Request[0|1] : Inport  Port=23
  n_Engine_Idle_Request[rpm] : Inport  Port=24
  Bus Creator : BusCreator  Inputs=24
  Enable_Trq_Decrease_Fast_ESP[0|1]_ : Subsystem
      mask Display: disp('')
  Enable_Trq_Increase_Fast_ESP[0|1]_ : Subsystem
      mask Display: disp('')
  Enable_Trq_Request_Extern1[0|1]_ : Subsystem
      mask Display: disp('')
  Enable_Trq_Request_Extern2[0|1]_ : Subsystem
      mask Display: disp('')
  Enable_n_Engine_Idle_Request[0|1]_ : Subsystem
      mask Display: disp('')
  Factor_Trq_Engine_Red[%]_ : Subsystem
      mask Display: disp('')
  Mode_StartButtonState[1Stim|2SoftECU]_ : Subsystem
      mask Display: disp('')
  Pos_AccPedal_Driver[%]_ : Subsystem
      mask Display: disp('')
  Reset_States[0|1]_ : Subsystem
      mask Display: disp('')
  State_StartButton[-1|0|1|2]_ : Subsystem
      mask Display: disp('')
  Sw_CrankShaft_Reset[0Disabled|1Enabled]_ : Subsystem
      mask Display: disp('')
  Sw_Ignition[0Off|1On]_ : Subsystem
      mask Display: disp('')
  Sw_ModelDeskPlottingInterface[0Disabled|1Enabled]_ : Subsystem
  Sw_ModelPortBlocks[0Disabled|1Enabled]_ : Subsystem
  Sw_StarterReq[0Off|1On]_ : Subsystem
      mask Display: disp('')
  Trq_Decrease_Request_Fast_ESP[Nm]_ : Subsystem
      mask Display: disp('')
  Trq_Increase_Request_Fast_ESP[Nm]_ : Subsystem
      mask Display: disp('')
  Trq_Request_Extern1[Nm]_ : Subsystem
      mask Display: disp('')
  Trq_Request_Extern2[Nm]_ : Subsystem
      mask Display: disp('')
  Trq_Request_ICE[Nm]_ : Subsystem
      mask Display: disp('')
  Vehicle_Topology[-2|-1|0|2]_ : Subsystem
      mask Display: disp('')
  n_Engine[rpm]_ : Subsystem
      mask Display: disp('')
  n_Engine_Idle_Request[rpm]_ : Subsystem
      mask Display: disp('')
  v_x_Vehicle[km|h]_ : Subsystem
      mask Display: disp('')
  Out : Outport  VectorParamsAs1DForOutWhenUnconnected=off
  wires:
  Sw_ModelDeskPlottingInterface[0Disabled|1Enabled]_/1(Out1) -> Bus Creator/2  "Sw_ModelDeskPlottingInterface[0Disabled|1Enabled]"
  Sw_ModelPortBlocks[0Disabled|1Enabled]_/1(Out1) -> Bus Creator/1  "Sw_ModelPortBlocks[0Disabled|1Enabled]"
  Sw_ModelDeskPlottingInterface[0Disabled|1Enabled]/1 -> Sw_ModelDeskPlottingInterface[0Disabled|1Enabled]_/1(In1)
  Sw_ModelPortBlocks[0Disabled|1Enabled]/1 -> Sw_ModelPortBlocks[0Disabled|1Enabled]_/1(In1)
  Bus Creator/1 -> Out/1  "ExternalModel"
  Trq_Request_ICE[Nm]/1 -> Trq_Request_ICE[Nm]_/1(In1)
  Trq_Request_ICE[Nm]_/1(Out1) -> Bus Creator/12  "Trq_Request_ICE[Nm]"
  Sw_Ignition[0Off|1On]_/1(Out1) -> Bus Creator/3  "Sw_Ignition[0Off|1On]"
  Sw_Ignition[0Off|1On]/1 -> Sw_Ignition[0Off|1On]_/1(In1)
  Sw_StarterReq[0Off|1On]/1 -> Sw_StarterReq[0Off|1On]_/1(In1)
  Sw_StarterReq[0Off|1On]_/1(Out1) -> Bus Creator/4  "Sw_StarterReq[0Off|1On]"
  Enable_Trq_Increase_Fast_ESP[0|1]_/1(Out1) -> Bus Creator/8  "Enable_Trq_Increase_Fast_ESP[0|1]"
  Trq_Increase_Request_Fast_ESP[Nm]_/1(Out1) -> Bus Creator/9  "Trq_Increase_Request_Fast_ESP[Nm]"
  Trq_Request_Extern1[Nm]_/1(Out1) -> Bus Creator/11  "Trq_Request_Extern1[Nm]"
  Enable_Trq_Request_Extern1[0|1]_/1(Out1) -> Bus Creator/10  "Enable_Trq_Request_Extern1[0|1]"
  Enable_Trq_Request_Extern1[0|1]/1 -> Enable_Trq_Request_Extern1[0|1]_/1(In1)
  Trq_Increase_Request_Fast_ESP[Nm]/1 -> Trq_Increase_Request_Fast_ESP[Nm]_/1(In1)
  Enable_Trq_Increase_Fast_ESP[0|1]/1 -> Enable_Trq_Increase_Fast_ESP[0|1]_/1(In1)
  Trq_Request_Extern1[Nm]/1 -> Trq_Request_Extern1[Nm]_/1(In1)
  Trq_Decrease_Request_Fast_ESP[Nm]_/1(Out1) -> Bus Creator/7  "Trq_Decrease_Request_Fast_ESP[Nm]"
  Enable_Trq_Decrease_Fast_ESP[0|1]_/1(Out1) -> Bus Creator/6  "Enable_Trq_Decrease_Fast_ESP[0|1]"
  Trq_Decrease_Request_Fast_ESP[Nm]/1 -> Trq_Decrease_Request_Fast_ESP[Nm]_/1(In1)
  Enable_Trq_Decrease_Fast_ESP[0|1]/1 -> Enable_Trq_Decrease_Fast_ESP[0|1]_/1(In1)
  Factor_Trq_Engine_Red[%]/1 -> Factor_Trq_Engine_Red[%]_/1(In1)
  Factor_Trq_Engine_Red[%]_/1(Out1) -> Bus Creator/5  "Factor_Trq_Engine_Red[%]"
  Trq_Request_Extern2[Nm]_/1(Out1) -> Bus Creator/22  "Trq_Request_Extern2[Nm]"
  Trq_Request_Extern2[Nm]/1 -> Trq_Request_Extern2[Nm]_/1(In1)
  Enable_Trq_Request_Extern2[0|1]/1 -> Enable_Trq_Request_Extern2[0|1]_/1(In1)
  Enable_Trq_Request_Extern2[0|1]_/1(Out1) -> Bus Creator/21  "Enable_Trq_Request_Extern2[0|1]"
  v_x_Vehicle[km|h]_/1(Out1) -> Bus Creator/18  "v_x_Vehicle[km|h]"
  Vehicle_Topology[-2|-1|0|2]/1 -> Vehicle_Topology[-2|-1|0|2]_/1(In1)
  State_StartButton[-1|0|1|2]/1 -> State_StartButton[-1|0|1|2]_/1(In1)
  Reset_States[0|1]_/1(Out1) -> Bus Creator/14  "Reset_States[0|1]"
  n_Engine[rpm]_/1(Out1) -> Bus Creator/13  "n_Engine[rpm]"
  Vehicle_Topology[-2|-1|0|2]_/1(Out1) -> Bus Creator/17  "Vehicle_Topology[-2|-1|0|2]"
  n_Engine[rpm]/1 -> n_Engine[rpm]_/1(In1)
  Pos_AccPedal_Driver[%]/1 -> Pos_AccPedal_Driver[%]_/1(In1)
  Pos_AccPedal_Driver[%]_/1(Out1) -> Bus Creator/15  "Pos_AccPedal_Driver[%]"
  v_x_Vehicle[km|h]/1 -> v_x_Vehicle[km|h]_/1(In1)
  Reset_States[0|1]/1 -> Reset_States[0|1]_/1(In1)
  State_StartButton[-1|0|1|2]_/1(Out1) -> Bus Creator/16  "State_StartButton[-1|0|1|2]"
  Mode_StartButtonState[1Stim|2SoftECU]_/1(Out1) -> Bus Creator/20  "Mode_StartButtonState[1Stim|2SoftECU]"
  Mode_StartButtonState[1Stim|2SoftECU]/1 -> Mode_StartButtonState[1Stim|2SoftECU]_/1(In1)
  Sw_CrankShaft_Reset[0Disabled|1Enabled]_/1(Out1) -> Bus Creator/19  "Sw_CrankShaft_Reset[0Disabled|1Enabled]"
  Sw_CrankShaft_Reset[0Disabled|1Enabled]/1 -> Sw_CrankShaft_Reset[0Disabled|1Enabled]_/1(In1)
  n_Engine_Idle_Request[rpm]/1 -> n_Engine_Idle_Request[rpm]_/1(In1)
  Enable_n_Engine_Idle_Request[0|1]_/1(Out1) -> Bus Creator/23  "Enable_n_Engine_Idle_Request[0|1]"
  n_Engine_Idle_Request[rpm]_/1(Out1) -> Bus Creator/24  "n_Engine_Idle_Request[rpm]"
  Enable_n_Engine_Idle_Request[0|1]/1 -> Enable_n_Engine_Idle_Request[0|1]_/1(In1)
